simulink model "SMTorqueControl"  (R2026a)
settings: Solver=FixedStepDiscrete  StopTime=1  FixedStep=Ts  EnableMultiTasking=on
PreLoadFcn:
  | if exist(fullfile(pwd, 'Ortak_Veri_ve_Parametreler'), 'dir'), addpath(fullfile(pwd, 'Ortak_Veri_ve_Parametreler')); end
  | if exist(fullfile(pwd, '..', 'Ortak_Veri_ve_Parametreler'), 'dir'), addpath(fullfile(pwd, '..', 'Ortak_Veri_ve_Parametreler')); end
  | if exist(fullfile(pwd, 'Mat_Dosyalari'), 'dir'), addpath(fullfile(pwd, 'Mat_Dosyalari')); end
  | SMTorqueControlData;
InitFcn:
  | if exist(fullfile(pwd, 'Ortak_Veri_ve_Parametreler'), 'dir'), addpath(fullfile(pwd, 'Ortak_Veri_ve_Parametreler')); end
  | if exist(fullfile(pwd, '..', 'Ortak_Veri_ve_Parametreler'), 'dir'), addpath(fullfile(pwd, '..', 'Ortak_Veri_ve_Parametreler')); end
  | if exist(fullfile(pwd, 'Mat_Dosyalari'), 'dir'), addpath(fullfile(pwd, 'Mat_Dosyalari')); end
  | SMTorqueControlData;
undefined symbols (not defined in the file): fsw, Ibase, Ifbase, L_base, Lad, Ld, Lq, p, Tbase, Ts, Tsi, VDC_VECT
libraries: nesl_utility x16, fl_lib x11, ee_lib x6, eeGeneralControl x3, eeTransforms x2, SignalEditorBlockLib x2, eeSmCurrentController x1, eeSmCurrentReferenceGen x1, eePwmGenerator x1, eePwmGeneratorTwoLevel x1, batteryecm_lib x1
Description:
  | SM Torque Control
settings Model: Creator=The MathWorks, Inc.  LastModifiedBy=Dogukan.kilinc
settings DataIOCC: MaxDataPoints=210000  SignalLoggingName=logsout_SMTorqueControl
settings SimscapeCC: SimscapeNominalValues="[{\"value\":\"1\",\"unit\":\"A\"},{\"value\":\"1\",\"unit\":\"bar\"},{\"value\":\"1\",\"unit\":\"cm^2\"},{\"value\":\"1\",\"unit\":\"cm^3/s\"},{\"value\":\"1\",\"unit\":\"kJ/kg\"},{\"value\":\"1\",\"unit\":\"kW\"},{\"value\":\"1\",\"unit\":\"l\"},{\"value\":\"1\",\"unit\":\"N\"},{\"value\":\"1\",\"unit\":\"N*m\"},{\"value\":\"1\",\"unit\":\"V\"}]"  SimscapeLogSimulationStatistics=on  SimscapeLogName=simlog_SMTorqueControl  SimscapeLogDataHistory=210000.0

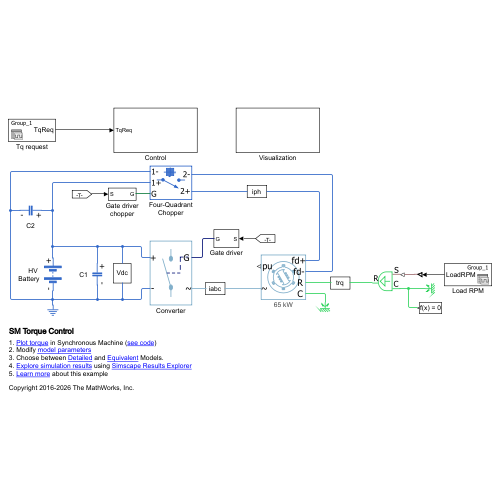
[thumbnail: Simulink's stored preview of the top-level diagram]
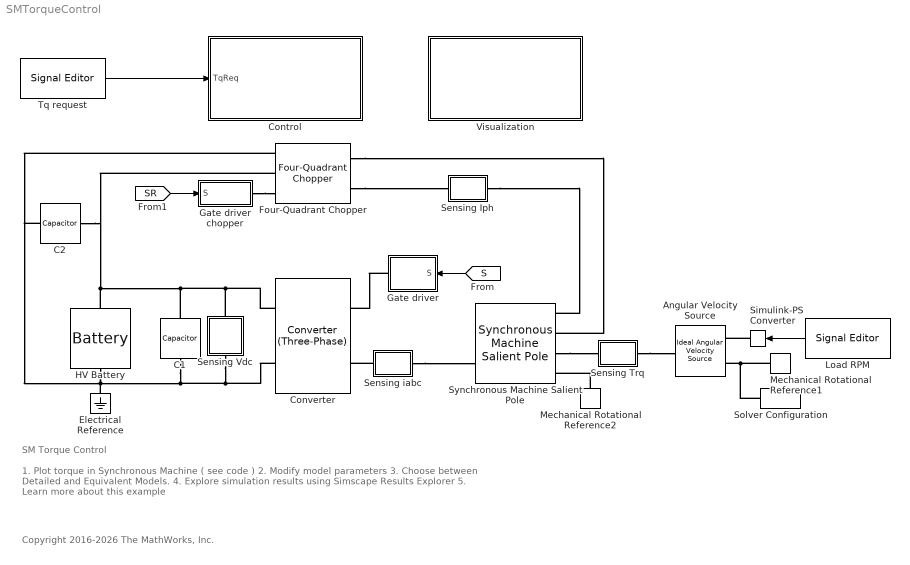
== system SMTorqueControl ==
  note: SM Torque Control
  note: 1. Plot torque in Synchronous Machine ( see code )
      | 2. Modify model parameters
      | 3. Choose between Detailed and Equivalent Models.
      | 4. Explore simulation results using Simscape Results Explorer
      | 5. Learn more about this example
  note: Copyright 2016-2026 The MathWorks, Inc.
  Angular Velocity Source : fl_lib/Mechanical/Mechanical Sources/Ideal Angular Velocity Source
  C1 : fl_lib/Electrical/Electrical Elements/Capacitor  c=Cdc F  r=1e-6 Ohm  g=0 1/Ohm  i_specify=off  i_priority=None  i=0 A  i_nominal_specify=off  i_nominal_value=1  i_nominal_unit=A  v_specify=off  v_priority=None  v=0 V  v_nominal_specify=off  v_nominal_value=1  v_nominal_unit=V  vc_specify=on  vc_priority=None  vc=Vnom V  vc_nominal_specify=off  vc_nominal_value=1  vc_nominal_unit=V
  C2 : fl_lib/Electrical/Electrical Elements/Capacitor  c=Cdc F  r=1e-6 Ohm  g=0 1/Ohm  i_specify=off  i_priority=None  i=0 A  i_nominal_specify=off  i_nominal_value=1  i_nominal_unit=A  v_specify=off  v_priority=None  v=0 V  v_nominal_specify=off  v_nominal_value=1  v_nominal_unit=V  vc_specify=on  vc_priority=None  vc=Vnom V  vc_nominal_specify=off  vc_nominal_value=1  vc_nominal_unit=V
  Control : Subsystem
  Converter : ee_lib/Semiconductors & Converters/Converters/Converter (Three-Phase)  port_option=ee.enum.threePhasePort.composite  fidelity_option=ee.enum.converters.fidelity.detailed  device_type=2  showThermalPort=false  K=0  Vth=0.5 V  Vgt=1 V  Vgt_off=-1 V  Ih=1 A  Vf=0.8 V  Ron=0.001 Ohm  Rds=0.001 Ohm  Goff=1e-5 1/Ohm  Eon_scalar=22.86e-3 J  Eoff_scalar=17.14e-3 J  Eoff_natural_commutation=10e-3 J  Voff=300 V  Iout_scalar=600 A  onCurrentMeasDelay=0 s  useCurrentFromPreviousCycle=false  useVoltageFromPreviousCycle=false  diode_param=2  diode_Vf=0.8 V  diode_Ron=0.001 Ohm  diode_Goff=1e-5 1/Ohm  diode_C=50 nF  diode_iRM=-235 A  diode_iF=300 A  diode_idot=-50 A/us  diode_trr_param=1  diode_trr_factor=3  diode_trr=15 us  diode_Qrr=1.5e+3 s*uA  diode_rec_loss_model=ee.enum.diode.reverseRecoveryModel.fixed  diode_ErecVal=0 J  diode_scaleWithIandV=false  diode_ErecMat=zeros(2, 3) J  diode_TjrecVec=[298.15, 398.15] K  diode_IfrecVec=[.1, 1, 10] A  diode_IrecVal=10 A  diode_VrecVal=10 V  diode_tFilter=1 / 1000 / 100 s  thermal_network_parameterization=ee.enum.thermalNetworkTopology.external  Rth=[.08, .5] K/W  Rth_Cauer=[.08, .1, .5] K/W  Rth_Foster=[.08, .14, .22, .16] K/W  thermal_mass_parameterization=ee.enum.thermalNetwork.timeconstant  thermal_mass=[.01, .5] J/K  thermal_mass_Cauer=[.01, .1, .5] J/K  thermal_mass_Foster=[.001, .005, .05, .5] J/K  thermal_time_constant=[.001, .2] s  thermal_time_constant_Cauer=[.001, .1, .2] s  thermal_time_constant_Foster=[7e-05, .0007, .01, .08] s  thermal_mass_initial_temperatures=[25, 25] degC  thermal_mass_initial_temperatures_Cauer=[25, 25, 25] degC  junction_thermal_mass=0.01 J/K  Tvec_initial_Foster=[25, 25, 25, 25] degC  snubber_type=0  Cs=1e-7 F  Rs=0.1 Ohm  Vce_loss=[0, 150, 300] V
  Electrical Reference : fl_lib/Electrical/Electrical Elements/Electrical Reference
  Four-Quadrant Chopper : ee_lib/Semiconductors & Converters/Converters/Four-Quadrant Chopper  fidelity_option=ee.enum.converters.fidelity.detailed  device_type=3  showThermalPort=false  Vgt=1 V  Vgt_off=-1 V  Ih=1 A  Vf=0.8 V  Ron=0.001 Ohm  Rds=0.001 Ohm  Goff=1e-5 1/Ohm  Vth=0.5 V  K=0  Eon_scalar=22.86e-3 J  Eoff_scalar=17.14e-3 J  Eoff_natural_commutation=10e-3 J  Voff=300 V  Iout_scalar=600 A  onCurrentMeasDelay=0 s  useCurrentFromPreviousCycle=false  useVoltageFromPreviousCycle=false  diode_param=2  diode_Vf=0.8 V  diode_Ron=0.001 Ohm  diode_Goff=1e-5 1/Ohm  diode_C=50 nF  diode_iRM=-235 A  diode_iF=300 A  diode_idot=-50 A/us  diode_trr_param=1  diode_trr_factor=3  diode_trr=15 us  diode_Qrr=1500 s*uA  diode_rec_loss_model=ee.enum.diode.reverseRecoveryModel.fixed  diode_ErecVal=0 J  diode_scaleWithIandV=false  diode_ErecMat=zeros(2, 3) J  diode_TjrecVec=[298.15, 398.15] K  diode_IfrecVec=[.1, 1, 10] A  diode_IrecVal=10 A  diode_VrecVal=10 V  diode_tFilter=1 / 1000 / 100 s  thermal_network_parameterization=ee.enum.thermalNetworkTopology.external  Rth=[.08, .5] K/W  Rth_Cauer=[.08, .1, .5] K/W  Rth_Foster=[.08, .14, .22, .16] K/W  thermal_mass_parameterization=ee.enum.thermalNetwork.timeconstant  thermal_mass=[.01, .5] J/K  thermal_mass_Cauer=[.01, .1, .5] J/K  thermal_mass_Foster=[.001, .005, .05, .5] J/K  thermal_time_constant=[.001, .2] s  thermal_time_constant_Cauer=[.001, .1, .2] s  thermal_time_constant_Foster=[7e-05, .0007, .01, .08] s  thermal_mass_initial_temperatures=[25, 25] degC  thermal_mass_initial_temperatures_Cauer=[25, 25, 25] degC  junction_thermal_mass=0.01 J/K  Tvec_initial_Foster=[25, 25, 25, 25] degC  snubber_type=0  Cs=1e-7 F  Rs=0.1 Ohm
  Gate driver : Subsystem
  Gate driver chopper : Subsystem
  HV Battery : batteryecm_lib/Battery  Vnom=Vnom V  prm_dir=1  R1_dis=2 Ohm  R1_ch=2 Ohm  R1=0.001 Ohm  prm_AH=1  AH=300 hr*A  V1=330 V  AH1=100 hr*A  prm_R2=1  R2=2000 Ohm  Tmeas=298.15 K  charge_measurement_port=simscape.enum.battery.enable.no  prm_dyn=1  Rp1=0.005 Ohm  tau1=30 s  Rp2=0.005 Ohm  tau2=30 s  Rp3=0.005 Ohm  tau3=30 s  Rp4=0.005 Ohm  tau4=30 s  Rp5=0.005 Ohm  tau5=30 s  prm_fade=1  N_fade=100  AH_fade=45 hr*A  R1_fade=2.02 Ohm  R1_ch_fade=2.02 Ohm  V1_fade=10.35 V  prm_age=1  prm_age_OCV=1  OCV_age=0.9  SOC_age=60  Tmeas_age=298.15 K  delta_time_age_vec=[0] d  temperature_age_vec=[273] K  OCV_scaling_age=2.2134e6  OCV_offset_age=1.632e6  temp_exp_age=0.515833569 V  t_exp_age=0.75  Vnom_T2=12 V  R1_T2=2.2 Ohm  R1_T2_dis=2.2 Ohm  R1_T2_ch=2.2 Ohm  V1_T2=11.4 V  R2_T2=2200 Ohm  Rp1_T2=0.005 Ohm  tau1_T2=30 s  Rp2_T2=0.005 Ohm  tau2_T2=30 s  Rp3_T2=0.005 Ohm  tau3_T2=30 s  Rp4_T2=0.005 Ohm  tau4_T2=30 s  Rp5_T2=0.005 Ohm  tau5_T2=30 s  Tmeas2=273.15 K  thermal_port=simscape.enum.thermaleffects.omit  thermal_mass=30000 J/K  i_specify=off  i_priority=None  i=0 A  i_nominal_specify=off  i_nominal_value=1  i_nominal_unit=A  v_specify=off  v_priority=None  v=0 V  v_nominal_specify=off  v_nominal_value=1  v_nominal_unit=V  charge_specify=on  charge_priority=High  charge=AH0 hr*A  charge_nominal_specify=off  charge_nominal_value=1  charge_nominal_unit=A*hr  num_cycles_specify=off  num_cycles_priority=High  num_cycles=0  num_cycles_nominal_specify=off  num_cycles_nominal_value=1  num_cycles_nominal_unit=1  temperature_specify=off  temperature_priority=High  temperature=298.15 K  temperature_nominal_specify=off  temperature_nominal_value=1  temperature_nominal_unit=K
  Load RPM : SignalEditorBlockLib/Signal Editor  FileName=SMTorqueControlLoadRPM.mat  ActiveScenario=Group_1  ActiveSignal=LoadRPM  IsBus=off  OutputBusObjectStr=Bus: BusObject  SampleTime=0  OutputAfterFinalValue=Extrapolation  Unit=inherit  PreserveSignalName=on  ApplySigPropsToAllScenarios=on  ApplySigPropsToAllSignals=off  SignalPropertySource=Dialog parameters
  Mechanical Rotational Reference1 : fl_lib/Mechanical/Rotational Elements/Mechanical Rotational Reference
  Mechanical Rotational Reference2 : fl_lib/Mechanical/Rotational Elements/Mechanical Rotational Reference
  Sensing Iph : Subsystem
      mask Display: disp('iph')
  Sensing Trq : Subsystem
      mask Display: disp('trq')
  Sensing Vdc : Subsystem
      mask Display: disp('Vdc')
  Sensing iabc : Subsystem
      mask Display: disp('iabc')
  Simulink-PS Converter : nesl_utility/Simulink-PS Converter  PhysicalDomain=network_engine_domain  SubClassName=ps_input  LeftPortType=input  RightPortType=output  PseudoPeriodic=off  Frequencies=[]  NoiseDistribution=none  NoiseParameters=[]  Unit=rpm  AffineConversion=off  FilteringAndDerivatives=zero  SimscapeFilterOrder=1  InputFilterTimeConstant=0.001  UdotUserProvided=1
  Solver Configuration : nesl_utility/Solver Configuration  PhysicalDomain=network_engine_domain  SubClassName=solver  LeftPortType=input  RightPortType=generic  Tones=[]  Harmonics=[]  SimulateNoise=off  Profile=off  UseLocalSampling=off  EnableSwitchedLinearOptims=on  FrequencyDomain=off  UseCCode=off  RelTol=0.001  AbsTol=1e-06  MinStep=1e-09  ToWorkspace=off  RevertToSquareIcSolve=off  NumHomotopyIterations=100  PhasorMode=off  PhasorModeNumHarmonics=1  ConsistencySolver=NEWTON_FTOL  CanonicalOrdering=UNORDERED  OptimizeIntermediates=UNOPTIMIZED  IndexReductionMethod=DerivativeReplacement  DoDC=off  ResidualTolerance=1e-9  ConsistencyTolSource=GLOBAL  ConsistencyAbsTol=0.001  ConsistencyRelTol=0.001  ConsistencyTolFactor=0.001  UseLocalSolver=on  LocalSolverChoice=NE_BACKWARD_EULER_ADVANCER  ResolveIndetEquations=on  FunctionEvalNumThread=1  LocalSolverSampleTime=Ts  DoFixedCost=on  MaxNonlinIter=4  MaxModeIter=2  ComputeImpulses=off  ImpulseIterations=2  LinearAlgebra=auto  LinearAlgebraNumThread=0  EquationFormulation=NE_TIME_EF  DelaysMemoryBudget=1024  AutomaticFiltering=on  FilteringTimeConstant=0.001  PartitionStorageMethod=AS_NEEDED  PartitionMemoryBudget=1024  PartitionMethod=FAST  MultibodyUseLocalSolver=off  MultibodyLocalSolverChoice=ODE1  MultibodyLocalSolverSampleTime=0.001
  Synchronous Machine Salient Pole : ee_lib/Electromechanical/Synchronous/Synchronous Machine Salient Pole  port_option=ee.enum.threePhasePort.composite  SRated=Pmax W  VRated=Vr V  FRated=fr Hz  nPolePairs=p  param_option=ee.enum.sm.parameterization.fundamental  fieldCircuitParameterization_option=2  baseEfd=272 V  baseIfd=Ifbase A  zero_sequence=ee.enum.park.zerosequence.exclude  axes_param=ee.enum.rotorangle.daxis  Ladu=Lad  Laqu=Laq  L0=L0  Ll=Ll  Ra=Rs  Lfd=Lfd  Rfd=Rfd  L1d=0.1  R1d=0.254  L1q=0.1567  R1q=0.328  Xl=0.15  Xd=1.05  Xq=0.7  X0=0.15  Xdd=0.35  Xddd=0.25  Xqdd=0.325  d_option=ee.enum.circuit.open  Td0d=5.25 s  Tdd=1.75 s  Td0dd=0.03 s  Tddd=0.0214 s  q_option=ee.enum.circuit.open  Tq0dd=0.05 s  Tqdd=0.0232 s  saturation_option=0  saturation_ifd=[0.0, 0.48, 0.76, 1.38, 1.79]  saturation_Vag=[0.0, 0.43, 0.59, 0.71, 0.76]  initialization_option=1  source_type=ee.enum.sm.load_flow_source_type.Swing  Vmag0=Vr V  Vang0=0 deg  Pt0=0 V*A  Qt0=0 V*A  minimum_pu=0.95  phase_search_range=[-30, 30] deg  gmin=1e-6 S  connection_option=ee.enum.Connection.wye  num_q_dampers=1  rotor_offset=-pi / 2 rad  pu_psid_specify=on  pu_psid_priority=High  pu_psid=0  pu_psid_nominal_specify=off  pu_psid_nominal_value=1  pu_psid_nominal_unit=1  pu_psiq_specify=on  pu_psiq_priority=High  pu_psiq=0  pu_psiq_nominal_specify=off  pu_psiq_nominal_value=1  pu_psiq_nominal_unit=1  pu_psifd_specify=on  pu_psifd_priority=High  pu_psifd=0  pu_psifd_nominal_specify=off  pu_psifd_nominal_value=1  pu_psifd_nominal_unit=1  pu_psi1d_specify=on  pu_psi1d_priority=High  pu_psi1d=0  pu_psi1d_nominal_specify=off  pu_psi1d_nominal_value=1  pu_psi1d_nominal_unit=1  pu_psi1q_specify=on  pu_psi1q_priority=High  pu_psi1q=0  pu_psi1q_nominal_specify=off  pu_psi1q_nominal_value=1  pu_psi1q_nominal_unit=1  angular_position_diff_specify=on  angular_position_diff_priority=High  angular_position_diff=-pi/2/p rad  angular_position_diff_nominal_specify=off  angular_position_diff_nominal_value=1  angular_position_diff_nominal_unit=deg  Tmeas=298.15 K  alpha=3.93e-3 1/K  stator_thermal_mass=100 J/K  rotor_thermal_mass=200 J/K  temperatureA_specify=off  temperatureA_priority=High  temperatureA=25 degC  temperatureA_nominal_specify=off  temperatureA_nominal_value=1  temperatureA_nominal_unit=degC  temperatureB_specify=off  temperatureB_priority=High  temperatureB=25 degC  temperatureB_nominal_specify=off  temperatureB_nominal_value=1  temperatureB_nominal_unit=degC  temperatureC_specify=off  temperatureC_priority=High  temperatureC=25 degC  temperatureC_nominal_specify=off  temperatureC_nominal_value=1  temperatureC_nominal_unit=degC  temperatureR_specify=off  temperatureR_priority=High  temperatureR=25 degC  temperatureR_nominal_specify=off  temperatureR_nominal_value=1  temperatureR_nominal_unit=degC
      settings: AttributesFormatString=65 kW
  Tq request : SignalEditorBlockLib/Signal Editor  FileName=SMTorqueControlTorqueRequest.mat  ActiveScenario=Group_1  ActiveSignal=TqReq  IsBus=off  OutputBusObjectStr=Bus: BusObject  SampleTime=0  OutputAfterFinalValue=Extrapolation  Unit=inherit  PreserveSignalName=on  ApplySigPropsToAllScenarios=on  ApplySigPropsToAllSignals=off  SignalPropertySource=Dialog parameters
  Visualization : Subsystem
  wires:
  [S] -> Gate driver/1(S)
  Load RPM/1 -> Simulink-PS Converter/1
  [SR] -> Gate driver chopper/1(S)
  Tq request/1 -> Control/1(TqReq)
  connections:
  Sensing Trq/RConn1 -- Angular Velocity Source/LConn1
  Converter/RConn2 -- Sensing Vdc/RConn1 -- Four-Quadrant Chopper/LConn3 -- C2/RConn1 -- HV Battery/RConn1 -- Electrical Reference/LConn1 -- C1/RConn1
  Converter/RConn1 -- Sensing Vdc/LConn1 -- Four-Quadrant Chopper/LConn2 -- C2/LConn1 -- HV Battery/LConn1 -- C1/LConn1
  Gate driver/RConn1 -- Converter/LConn1
  Simulink-PS Converter/RConn1 -- Angular Velocity Source/RConn1
  Synchronous Machine Salient Pole/LConn3 -- Sensing Trq/LConn1
  Mechanical Rotational Reference1/LConn1 -- Solver Configuration/RConn1 -- Angular Velocity Source/RConn2
  Four-Quadrant Chopper/RConn1 -- Sensing Iph/LConn1
  Four-Quadrant Chopper/RConn2 -- Synchronous Machine Salient Pole/LConn2
  Sensing Iph/RConn1 -- Synchronous Machine Salient Pole/LConn1
  Sensing iabc/LConn1 -- Converter/LConn2
  Sensing iabc/RConn1 -- Synchronous Machine Salient Pole/RConn2
  Gate driver chopper/RConn1 -- Four-Quadrant Chopper/LConn1
  Mechanical Rotational Reference2/LConn1 -- Synchronous Machine Salient Pole/LConn4

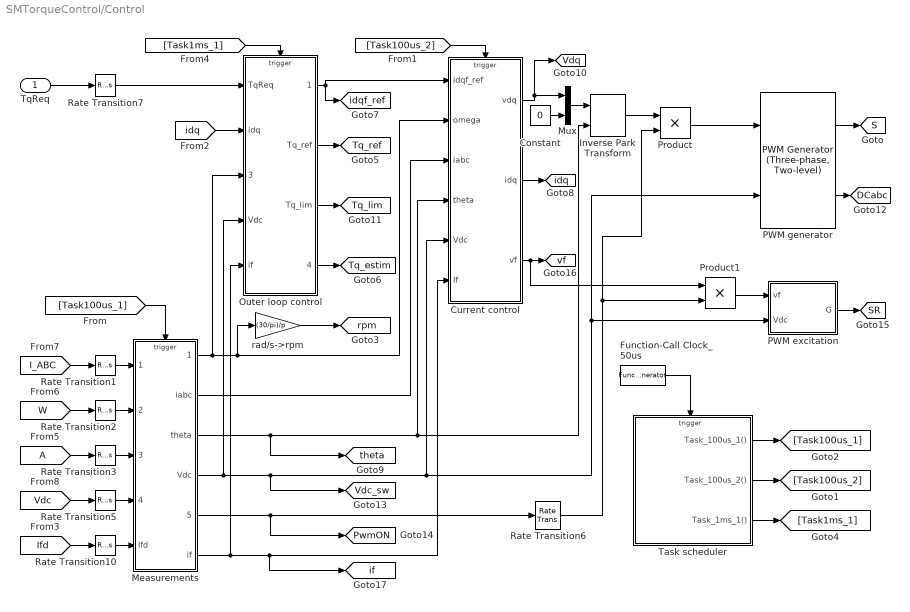
== system SMTorqueControl/Control ==
  TqReq : Inport
  Constant : Constant  Value=0  SampleTime=-1
  Current control : Subsystem
  From5 : From  TagVisibility=global
  Function-Call Clock_50us : FunctionCallGenerator  SampleTime=5e-5
  Inverse Park Transform : eeTransforms/Inverse Park Transform  AxisAlignment=Q-axis  PowerInvariant=off
  Measurements : Subsystem
  Mux : Mux  Inputs=2
  Outer loop control : Subsystem
  PWM excitation : Subsystem
  PWM generator : eePwmGeneratorTwoLevel/PWM Generator (Three-phase, Two-level)  PWMMode=Continuous PWM (CPWM)  CPWMMode=SVM: space vector modulation  DPWMMode=60 DPWM: 60 degree discontinuous PWM  fsw=fsw  Ts=Ts
  Product : Product
  Product1 : Product
  Rate Transition{1..3,5..7,10} (7 alike) : RateTransition
  Task scheduler : Stateflow chart  TreatAsAtomicUnit=on
  rad/s->rpm : Gain  Gain=(30/pi)/p
  tag scope: DCabc=global, PwmON=global, S=global, SR=global, Tq_estim=global, Tq_lim=global, Tq_ref=global, Vdc_sw=global, Vdq=global, idq=global, idqf_ref=global, if=global, rpm=global, theta=global, vf=global
  wires:
  [Ifd] -> Rate Transition10/1
  [W] -> Rate Transition2/1
  [idq] -> Outer loop control/2(idq)
  [Task100us_1] -> Measurements/Trigger
  Measurements/5(PwmON) -> Rate Transition6/1, [PwmON]
  Rate Transition1/1 -> Measurements/1(iabc_m)
  PWM generator/2 -> [DCabc]
  [I_ABC] -> Rate Transition1/1
  Rate Transition6/1 -> Product1/2, Product/2
  [Task100us_2] -> Current control/Trigger
  Measurements/2(iabc) -> Current control/3(iabc)
  Outer loop control/4(Tq_estim) -> [Tq_estim]
  Current control/3(vf) -> Product1/1, [vf]
  Measurements/1(omega) -> rad/s->rpm/1, Current control/2(omega), Outer loop control/3(omega)
  rad/s->rpm/1 -> [rpm]
  Current control/2(idq) -> [idq]
  Rate Transition10/1 -> Measurements/5(Ifd)
  Task scheduler/2(Task_100us_2()) -> [Task100us_2]
  From5/1 -> Rate Transition3/1
  Measurements/3(theta) -> [theta], Inverse Park Transform/2, Current control/4(theta)
  Outer loop control/2(Tq_ref) -> [Tq_ref]
  Task scheduler/1(Task_100us_1()) -> [Task100us_1]
  [Task1ms_1] -> Outer loop control/Trigger
  Rate Transition2/1 -> Measurements/2(omega_m)
  Task scheduler/3(Task_1ms_1()) -> [Task1ms_1]
  TqReq/1 -> Rate Transition7/1
  Measurements/4(Vdc) -> [Vdc_sw], PWM generator/2, PWM excitation/2(Vdc), Current control/5(Vdc), Outer loop control/4(Vdc)
  [Vdc] -> Rate Transition5/1
  Rate Transition5/1 -> Measurements/4(Vdc_m)
  PWM generator/1 -> [S]
  Rate Transition3/1 -> Measurements/3(theta_m)
  Outer loop control/3(Tq_lim) -> [Tq_lim]
  Measurements/6(if) -> [if], Current control/6(If), Outer loop control/5(if)
  PWM excitation/1(G) -> [SR]
  Function-Call Clock_50us/1 -> Task scheduler/Trigger
  Rate Transition7/1 -> Outer loop control/1(TqReq)
  Outer loop control/1(idqf_ref) -> Current control/1(idqf_ref), [idqf_ref]
  Constant/1 -> Mux/2
  Mux/1 -> Inverse Park Transform/1
  Current control/1(vdq) -> [Vdq], Mux/1
  Product/1 -> PWM generator/1
  Inverse Park Transform/1 -> Product/1
  Product1/1 -> PWM excitation/1(vf)

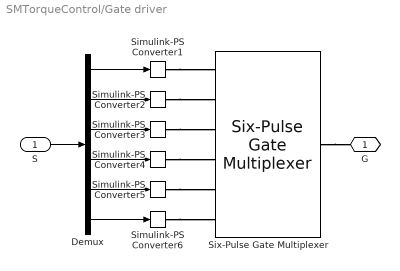
== system SMTorqueControl/Gate driver ==
  S : Inport
  Demux : Demux  Outputs=6
  Simulink-PS Converter{1..6} (6 alike) : nesl_utility/Simulink-PS Converter  PhysicalDomain=network_engine_domain  SubClassName=ps_input  LeftPortType=input  RightPortType=output  PseudoPeriodic=off  Frequencies=[]  NoiseDistribution=none  NoiseParameters=[]  Unit=1  AffineConversion=off  FilteringAndDerivatives=zero  SimscapeFilterOrder=1  InputFilterTimeConstant=0.001  UdotUserProvided=1
  Six-Pulse Gate Multiplexer : ee_lib/Semiconductors & Converters/Converters/Six-Pulse Gate Multiplexer  port_option=ee.enum.controlport.ps
  G : PMIOPort  Side=Right
  wires:
  Demux/1 -> Simulink-PS Converter1/1
  S/1 -> Demux/1
  Demux/4 -> Simulink-PS Converter4/1
  Demux/2 -> Simulink-PS Converter2/1
  Demux/3 -> Simulink-PS Converter3/1
  Demux/5 -> Simulink-PS Converter5/1
  Demux/6 -> Simulink-PS Converter6/1
  connections:
  Six-Pulse Gate Multiplexer/RConn1 -- G/RConn1
  Simulink-PS Converter1/RConn1 -- Six-Pulse Gate Multiplexer/LConn1
  Simulink-PS Converter3/RConn1 -- Six-Pulse Gate Multiplexer/LConn3
  Simulink-PS Converter5/RConn1 -- Six-Pulse Gate Multiplexer/LConn5
  Simulink-PS Converter6/RConn1 -- Six-Pulse Gate Multiplexer/LConn6
  Simulink-PS Converter4/RConn1 -- Six-Pulse Gate Multiplexer/LConn4
  Simulink-PS Converter2/RConn1 -- Six-Pulse Gate Multiplexer/LConn2

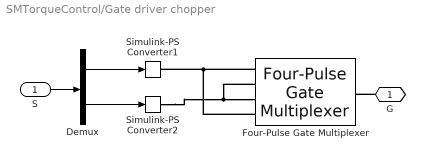
== system SMTorqueControl/Gate driver chopper ==
  S : Inport
  Demux : Demux  Outputs=2
  Four-Pulse Gate Multiplexer : ee_lib/Semiconductors & Converters/Converters/Four-Pulse Gate Multiplexer  port_option=ee.enum.controlport.ps
  Simulink-PS Converter1 : nesl_utility/Simulink-PS Converter  PhysicalDomain=network_engine_domain  SubClassName=ps_input  LeftPortType=input  RightPortType=output  PseudoPeriodic=off  Frequencies=[]  NoiseDistribution=none  NoiseParameters=[]  Unit=1  AffineConversion=off  FilteringAndDerivatives=zero  SimscapeFilterOrder=1  InputFilterTimeConstant=0.001  UdotUserProvided=1
  Simulink-PS Converter2 : nesl_utility/Simulink-PS Converter  PhysicalDomain=network_engine_domain  SubClassName=ps_input  LeftPortType=input  RightPortType=output  PseudoPeriodic=off  Frequencies=[]  NoiseDistribution=none  NoiseParameters=[]  Unit=1  AffineConversion=off  FilteringAndDerivatives=zero  SimscapeFilterOrder=1  InputFilterTimeConstant=0.001  UdotUserProvided=1
  G : PMIOPort  Side=Right
  wires:
  Demux/2 -> Simulink-PS Converter2/1
  S/1 -> Demux/1
  Demux/1 -> Simulink-PS Converter1/1
  connections:
  Simulink-PS Converter2/RConn1 -- Four-Pulse Gate Multiplexer/LConn2 -- Four-Pulse Gate Multiplexer/LConn3
  Four-Pulse Gate Multiplexer/LConn1 -- Four-Pulse Gate Multiplexer/LConn4 -- Simulink-PS Converter1/RConn1
  G/RConn1 -- Four-Pulse Gate Multiplexer/RConn1

== system SMTorqueControl/Sensing Iph ==
  Current Sensor : fl_lib/Electrical/Electrical Sensors/Current Sensor
  PS-Simulink Converter : nesl_utility/PS-Simulink Converter  PhysicalDomain=network_engine_domain  SubClassName=ps_output  LeftPortType=input  RightPortType=output  PseudoPeriodic=off  Frequencies=[]  VectorFormat=1-D array  Unit=1  AffineConversion=off
  + : PMIOPort  Side=Left
  - : PMIOPort  Port=2  Side=Right
  tag scope: Ifd=global
  wires:
  PS-Simulink Converter/1 -> [Ifd]
  connections:
  Current Sensor/LConn1 -- +/RConn1
  Current Sensor/RConn2 -- -/RConn1
  PS-Simulink Converter/LConn1 -- Current Sensor/RConn1

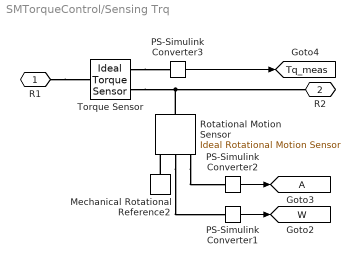
== system SMTorqueControl/Sensing Trq ==
  Goto3 : Goto  TagVisibility=global
  Mechanical Rotational Reference2 : fl_lib/Mechanical/Rotational Elements/Mechanical Rotational Reference
  PS-Simulink Converter1 : nesl_utility/PS-Simulink Converter  PhysicalDomain=network_engine_domain  SubClassName=ps_output  LeftPortType=input  RightPortType=output  PseudoPeriodic=off  Frequencies=[]  VectorFormat=1-D array  Unit=rad/s  AffineConversion=off
  PS-Simulink Converter2 : nesl_utility/PS-Simulink Converter  PhysicalDomain=network_engine_domain  SubClassName=ps_output  LeftPortType=input  RightPortType=output  PseudoPeriodic=off  Frequencies=[]  VectorFormat=1-D array  Unit=rad  AffineConversion=off
  PS-Simulink Converter3 : nesl_utility/PS-Simulink Converter  PhysicalDomain=network_engine_domain  SubClassName=ps_output  LeftPortType=input  RightPortType=output  PseudoPeriodic=off  Frequencies=[]  VectorFormat=1-D array  Unit=N*m  AffineConversion=off
  Rotational Motion Sensor : fl_lib/Mechanical/Mechanical Sensors/Ideal Rotational Motion Sensor  reference=foundation.enum.MeasurementReference.difference  acceleration_port=false  velocity_port=true  position_port=true  wrap_angle=simscape.enum.onoff.off  offset=0 deg
  Torque Sensor : fl_lib/Mechanical/Mechanical Sensors/Ideal Torque Sensor
  R1 : PMIOPort  Side=Left
  R2 : PMIOPort  Port=2  Side=Right
  tag scope: Tq_meas=global, W=global
  wires:
  PS-Simulink Converter1/1 -> [W]
  PS-Simulink Converter2/1 -> Goto3/1
  PS-Simulink Converter3/1 -> [Tq_meas]
  connections:
  Rotational Motion Sensor/LConn1 -- Torque Sensor/RConn1 -- R2/RConn1
  Torque Sensor/RConn2 -- PS-Simulink Converter3/LConn1
  Rotational Motion Sensor/RConn2 -- PS-Simulink Converter1/LConn1
  Rotational Motion Sensor/RConn3 -- PS-Simulink Converter2/LConn1
  Mechanical Rotational Reference2/LConn1 -- Rotational Motion Sensor/RConn1
  R1/RConn1 -- Torque Sensor/LConn1

== system SMTorqueControl/Sensing Vdc ==
  PS-Simulink Converter4 : nesl_utility/PS-Simulink Converter  PhysicalDomain=network_engine_domain  SubClassName=ps_output  LeftPortType=input  RightPortType=output  PseudoPeriodic=off  Frequencies=[]  VectorFormat=1-D array  Unit=V  AffineConversion=off
  Voltage Sensor : fl_lib/Electrical/Electrical Sensors/Voltage Sensor
  + : PMIOPort  Side=Left
  - : PMIOPort  Port=2  Side=Right
  tag scope: Vdc=global
  wires:
  PS-Simulink Converter4/1 -> [Vdc]
  connections:
  Voltage Sensor/LConn1 -- +/RConn1
  Voltage Sensor/RConn2 -- -/RConn1
  PS-Simulink Converter4/LConn1 -- Voltage Sensor/RConn1

== system SMTorqueControl/Sensing iabc ==
  Current Sensor : ee_lib/Sensors & Transducers/Current Sensor (Three-Phase)  port_option=ee.enum.threePhasePort.composite
  PS-Simulink Converter : nesl_utility/PS-Simulink Converter  PhysicalDomain=network_engine_domain  SubClassName=ps_output  LeftPortType=input  RightPortType=output  PseudoPeriodic=off  Frequencies=[]  VectorFormat=1-D array  Unit=A  AffineConversion=off
  1 : PMIOPort  Side=Left
  2 : PMIOPort  Port=2  Side=Right
  tag scope: I_ABC=global
  wires:
  PS-Simulink Converter/1 -> [I_ABC]
  connections:
  1/RConn1 -- Current Sensor/LConn1
  2/RConn1 -- Current Sensor/RConn2
  Current Sensor/RConn1 -- PS-Simulink Converter/LConn1

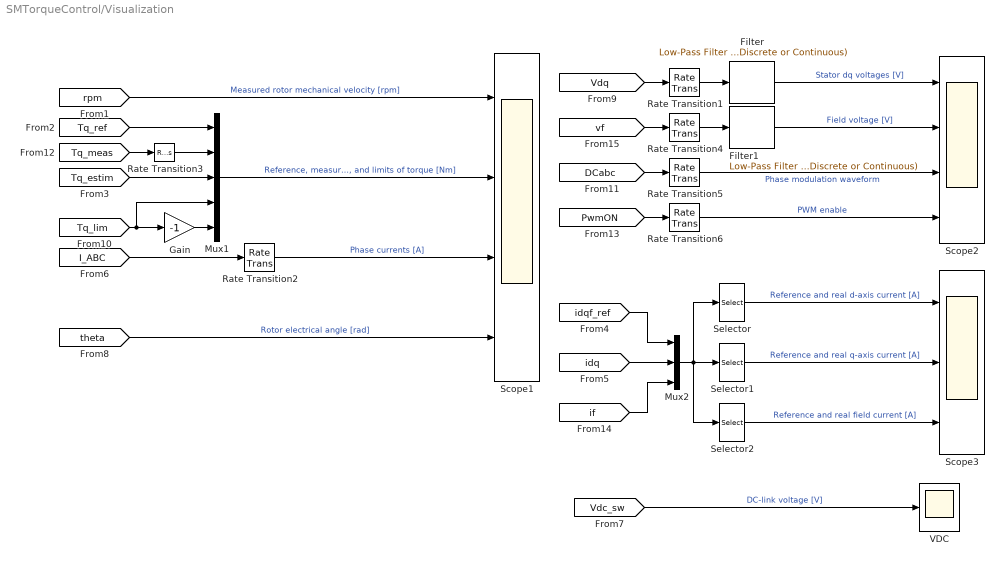
== system SMTorqueControl/Visualization ==
  Filter : eeGeneralControl/Low-Pass Filter (Discrete or Continuous)  K=1  T=0.05  B=inf  A=-inf  init_option=Inherited from block input  x0=0  Ts=Tsi
  Filter1 : eeGeneralControl/Low-Pass Filter (Discrete or Continuous)  K=1  T=0.05  B=inf  A=-inf  init_option=Inherited from block input  x0=0  Ts=Tsi
  Gain : Gain  Gain=-1
  Mux1 : Mux  Inputs=5
  Mux2 : Mux  Inputs=3
  Rate Transition{1,4..6} (4 alike) : RateTransition  OutPortSampleTime=Tsi
  Rate Transition2 : RateTransition
  Rate Transition3 : RateTransition
  Scope1 : Scope  NumInputPorts=4
      settings: ActiveDisplayYMinimum=-250  ActiveDisplayYMaximum=2250  DataLoggingSaveFormat=Array
  Scope2 : Scope  NumInputPorts=4
      settings: ActiveDisplayYMinimum=-110.23475  ActiveDisplayYMaximum=89.83125  DataLoggingVariableName=ScopeData3  DataLoggingSaveFormat=Array
  "Scope3 " : Scope  NumInputPorts=3
      settings: ActiveDisplayYMinimum=-147.62964  ActiveDisplayYMaximum=49.34388  DataLoggingVariableName=ScopeData2  DataLoggingSaveFormat=Array
  Selector : Selector  InputPortWidth=6  IndexOptions=Index vector (dialog)  Indices=[1 4]  OutputSizes=1
  Selector1 : Selector  InputPortWidth=6  IndexOptions=Index vector (dialog)  Indices=[2 5]  OutputSizes=1
  Selector2 : Selector  InputPortWidth=6  IndexOptions=Index vector (dialog)  Indices=[3 6]  OutputSizes=1
  VDC : Scope
      settings: ActiveDisplayYMinimum=-43.65366  ActiveDisplayYMaximum=392.90021  DataLoggingSaveFormat=Array
  wires:
  [if] -> Mux2/3
  Filter/1 -> Scope2/1  "Stator dq voltages [V]"
  [DCabc] -> Rate Transition5/1
  Rate Transition3/1 -> Mux1/2
  [Tq_ref] -> Mux1/1
  [Vdc_sw] -> VDC/1  "DC-link voltage [V]"
  [PwmON] -> Rate Transition6/1
  [rpm] -> Scope1/1  "Measured rotor mechanical velocity [rpm]"
  [Tq_meas] -> Rate Transition3/1
  Rate Transition2/1 -> Scope1/3  "Phase currents [A]"
  Mux2/1 -> Selector/1, Selector2/1, Selector1/1
  [Tq_estim] -> Mux1/3
  [idqf_ref] -> Mux2/1
  [idq] -> Mux2/2
  [Tq_lim] -> Gain/1, Mux1/4
  Filter1/1 -> Scope2/2  "Field voltage [V]"
  [theta] -> Scope1/4  "Rotor electrical angle [rad]"
  Gain/1 -> Mux1/5
  [I_ABC] -> Rate Transition2/1
  Mux1/1 -> Scope1/2  "Reference, measured, estim, and limits of torque [Nm]"
  Selector1/1 -> "Scope3 "/2  "Reference and real q-axis current [A]"
  Selector/1 -> "Scope3 "/1  "Reference and real d-axis current [A]"
  Selector2/1 -> "Scope3 "/3  "Reference and real field current [A]"
  Rate Transition4/1 -> Filter1/1
  Rate Transition1/1 -> Filter/1
  [Vdq] -> Rate Transition1/1
  [vf] -> Rate Transition4/1
  Rate Transition5/1 -> Scope2/3  "Phase modulation waveform"
  Rate Transition6/1 -> Scope2/4  "PWM enable"

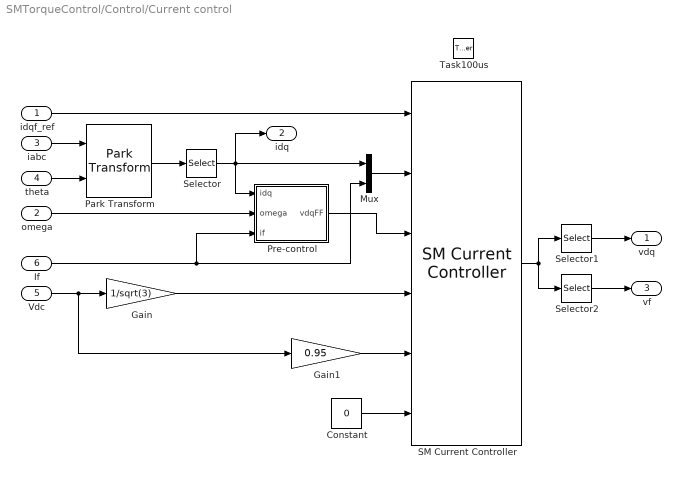
== system SMTorqueControl/Control/Current control ==
  idqf_ref : Inport
  omega : Inport  Port=2
  iabc : Inport  Port=3
  theta : Inport  Port=4
  Vdc : Inport  Port=5
  If : Inport  Port=6
  Task100us : TriggerPort  TriggerType=function-call  VariantControl=Variant  PortDimensions=1
  Constant : Constant  Value=0  SampleTime=-1
  Gain : Gain  Gain=1/sqrt(3)
  Gain1 : Gain  Gain=0.95
  Mux : Mux  Inputs=2
  Park Transform : eeTransforms/Park Transform  AxisAlignment=Q-axis  PowerInvariant=off
  Pre-control : Subsystem
  SM Current Controller : eeSmCurrentController/SM Current Controller  Ts=-1  Tsd=Tsi  AxisPrio=Q-axis  ActZC=on  ActFF=on  Kp_id=Kp_id  Ki_id=Ki_id  Kaw_id=Kaw_id  Kp_iq=Kp_iq  Ki_iq=Ki_iq  Kaw_iq=Kaw_iq  Kp_if=Kp_if  Ki_if=Ki_if  Kaw_if=Kaw_if
  Selector : Selector  InputPortWidth=3  IndexOptions=Index vector (dialog)  Indices=[1 2]  OutputSizes=1
  Selector1 : Selector  InputPortWidth=3  IndexOptions=Index vector (dialog)  Indices=[1 2]  OutputSizes=1
  Selector2 : Selector  InputPortWidth=3  IndexOptions=Index vector (dialog)  Indices=3  OutputSizes=1
  vdq : Outport  VectorParamsAs1DForOutWhenUnconnected=off
  idq : Outport  Port=2  VectorParamsAs1DForOutWhenUnconnected=off
  vf : Outport  Port=3  VectorParamsAs1DForOutWhenUnconnected=off
  wires:
  iabc/1 -> Park Transform/1
  Park Transform/1 -> Selector/1
  theta/1 -> Park Transform/2
  idqf_ref/1 -> SM Current Controller/1
  Selector/1 -> Mux/1, idq/1, Pre-control/1(idq)
  Pre-control/1(vdqFF) -> SM Current Controller/3
  Vdc/1 -> Gain1/1, Gain/1
  omega/1 -> Pre-control/2(omega)
  If/1 -> Pre-control/3(if), Mux/2
  Gain/1 -> SM Current Controller/4
  Gain1/1 -> SM Current Controller/5
  Constant/1 -> SM Current Controller/6
  SM Current Controller/1 -> Selector2/1, Selector1/1
  Selector1/1 -> vdq/1
  Selector2/1 -> vf/1
  Mux/1 -> SM Current Controller/2

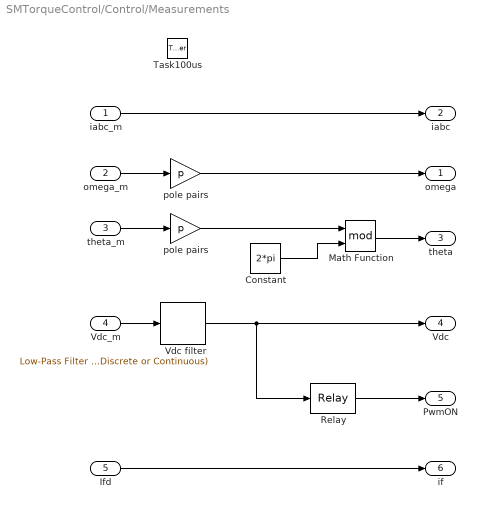
== system SMTorqueControl/Control/Measurements ==
  iabc_m : Inport
  omega_m : Inport  Port=2
  theta_m : Inport  Port=3
  Vdc_m : Inport  Port=4
  Ifd : Inport  Port=5
  Task100us : TriggerPort  TriggerType=function-call  VariantControl=Variant  PortDimensions=1
  Constant : Constant  Value=2*pi  SampleTime=-1
  Math Function : Math  Operator=mod  SignedPower=on
  Relay : Relay  OnSwitchValue=VDC_VECT(1)  OffSwitchValue=0.5*VDC_VECT(1)
  Vdc filter : eeGeneralControl/Low-Pass Filter (Discrete or Continuous)  K=1  T=0.005  B=inf  A=-inf  init_option=Inherited from block input  x0=0  Ts=-1
  pole pairs : Gain  Gain=p
  "pole pairs " : Gain  Gain=p
  omega : Outport  VectorParamsAs1DForOutWhenUnconnected=off
  iabc : Outport  Port=2  VectorParamsAs1DForOutWhenUnconnected=off
  theta : Outport  Port=3  VectorParamsAs1DForOutWhenUnconnected=off
  Vdc : Outport  Port=4  VectorParamsAs1DForOutWhenUnconnected=off
  PwmON : Outport  Port=5  VectorParamsAs1DForOutWhenUnconnected=off
  if : Outport  Port=6  VectorParamsAs1DForOutWhenUnconnected=off
  wires:
  pole pairs/1 -> omega/1
  Vdc_m/1 -> Vdc filter/1
  theta_m/1 -> "pole pairs "/1
  omega_m/1 -> pole pairs/1
  iabc_m/1 -> iabc/1
  "pole pairs "/1 -> Math Function/1
  Constant/1 -> Math Function/2
  Math Function/1 -> theta/1
  Relay/1 -> PwmON/1
  Vdc filter/1 -> Relay/1, Vdc/1
  Ifd/1 -> if/1

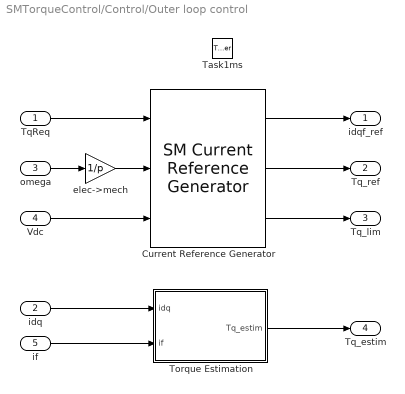
== system SMTorqueControl/Control/Outer loop control ==
  TqReq : Inport
  idq : Inport  Port=2
  omega : Inport  Port=3
  Vdc : Inport  Port=4
  if : Inport  Port=5
  Task1ms : TriggerPort  TriggerType=function-call  VariantControl=Variant  PortDimensions=1
  Current Reference Generator : eeSmCurrentReferenceGen/SM Current Reference Generator  Vnom=Vnom  Pmax=Pmax  Tmax=Tbase  ifmax=Ifbase  Ts=-1  RefType=Lookup-table based  rpmVec=RPM_VECT  TqVec=TQ_VECT  VdcVec=VDC_VECT  idMatrix=ID_MAP  iqMatrix=IQ_MAP  ifMatrix=IF_MAP  Kt=0.0375
  Torque Estimation : Subsystem
  elec->mech : Gain  Gain=1/p
  idqf_ref : Outport  VectorParamsAs1DForOutWhenUnconnected=off
  Tq_ref : Outport  Port=2  VectorParamsAs1DForOutWhenUnconnected=off
  Tq_lim : Outport  Port=3  VectorParamsAs1DForOutWhenUnconnected=off
  Tq_estim : Outport  Port=4  VectorParamsAs1DForOutWhenUnconnected=off
  wires:
  Torque Estimation/1(Tq_estim) -> Tq_estim/1
  idq/1 -> Torque Estimation/1(idq)
  if/1 -> Torque Estimation/2(if)
  Current Reference Generator/1 -> idqf_ref/1
  elec->mech/1 -> Current Reference Generator/2
  Current Reference Generator/3 -> Tq_lim/1
  Vdc/1 -> Current Reference Generator/3
  TqReq/1 -> Current Reference Generator/1
  omega/1 -> elec->mech/1
  Current Reference Generator/2 -> Tq_ref/1

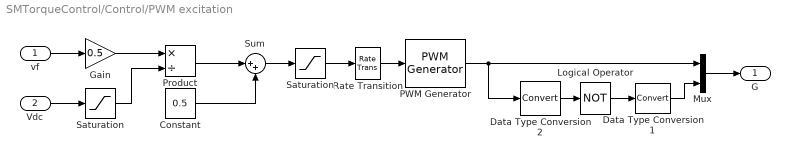
== system SMTorqueControl/Control/PWM excitation ==
  vf : Inport
  Vdc : Inport  Port=2
  Constant : Constant  Value=0.5  SampleTime=-1
  Data Type Conversion1 : DataTypeConversion  SaturateOnIntegerOverflow=off  RndMeth=Floor
  Data Type Conversion2 : DataTypeConversion  SaturateOnIntegerOverflow=off  RndMeth=Floor
  Gain : Gain  Gain=0.5
  Logical Operator : Logic  Operator=NOT  AllPortsSameDT=off  OutDataTypeStr=boolean
  Mux : Mux  Inputs=2
  PWM Generator : eePwmGenerator/PWM Generator  CarrCount=Up  Tper=1/fsw  Tdelay=0  Ts=Ts
  Product : Product  Inputs=*/
  Rate Transition : RateTransition
  Saturation : Saturate  UpperLimit=inf  LowerLimit=1
  "Saturation " : Saturate  UpperLimit=1  LowerLimit=0
  Sum : Sum  Inputs=|++
  G : Outport  VectorParamsAs1DForOutWhenUnconnected=off
  wires:
  vf/1 -> Gain/1
  Vdc/1 -> Saturation/1
  Saturation/1 -> Product/2
  Constant/1 -> Sum/2
  Sum/1 -> "Saturation "/1
  "Saturation "/1 -> Rate Transition/1
  Gain/1 -> Product/1
  Product/1 -> Sum/1
  Rate Transition/1 -> PWM Generator/1
  Data Type Conversion1/1 -> Mux/2
  PWM Generator/1 -> Data Type Conversion2/1, Mux/1
  Mux/1 -> G/1
  Data Type Conversion2/1 -> Logical Operator/1
  Logical Operator/1 -> Data Type Conversion1/1

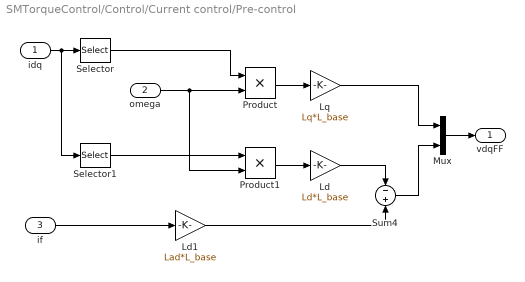
== system SMTorqueControl/Control/Current control/Pre-control ==
  idq : Inport
  omega : Inport  Port=2
  if : Inport  Port=3
  Ld : Gain  Gain=Ld*L_base
  Ld1 : Gain  Gain=Lad*L_base
  Lq : Gain  Gain=Lq*L_base
  Mux : Mux  Inputs=2
  Product : Product
  Product1 : Product
  Selector : Selector  InputPortWidth=2  IndexOptions=Index vector (dialog)  Indices=2  OutputSizes=1
  Selector1 : Selector  InputPortWidth=2  IndexOptions=Index vector (dialog)  Indices=1  OutputSizes=1
  Sum4 : Sum  Inputs=-+
  vdqFF : Outport  VectorParamsAs1DForOutWhenUnconnected=off
  wires:
  idq/1 -> Selector1/1, Selector/1
  Mux/1 -> vdqFF/1
  Selector1/1 -> Product1/1
  omega/1 -> Product1/2, Product/2
  Ld/1 -> Sum4/1
  if/1 -> Ld1/1
  Sum4/1 -> Mux/2
  Lq/1 -> Mux/1
  Ld1/1 -> Sum4/2
  Selector/1 -> Product/1
  Product1/1 -> Ld/1
  Product/1 -> Lq/1

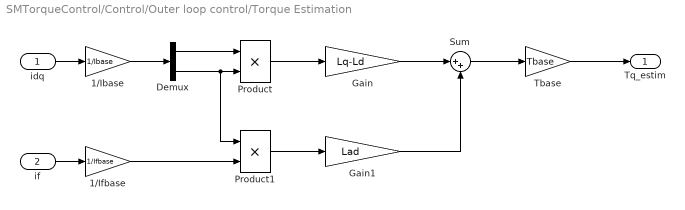
== system SMTorqueControl/Control/Outer loop control/Torque Estimation ==
  idq : Inport
  if : Inport  Port=2
  1/Ibase : Gain  Gain=1/Ibase
  1/Ifbase : Gain  Gain=1/Ifbase
  Demux : Demux  Outputs=2
  Gain : Gain  Gain=Lq-Ld
  Gain1 : Gain  Gain=Lad
  Product : Product
  Product1 : Product
  Sum : Sum  Inputs=|++
  Tbase : Gain  Gain=Tbase
  Tq_estim : Outport  VectorParamsAs1DForOutWhenUnconnected=off
  wires:
  idq/1 -> 1/Ibase/1
  Demux/1 -> Product/1
  Product/1 -> Gain/1
  Gain/1 -> Sum/1
  Demux/2 -> Product1/1, Product/2
  Product1/1 -> Gain1/1
  Sum/1 -> Tbase/1
  if/1 -> 1/Ifbase/1
  1/Ifbase/1 -> Product1/2
  1/Ibase/1 -> Demux/1
  Tbase/1 -> Tq_estim/1
  Gain1/1 -> Sum/2

== stateflow chart SMTorqueControl/Control/Task scheduler ==
  (default) -> (junction 23) : CLK_50us
  (junction 23) -> (junction 17)
  (junction 17) -> (junction 22) [order 2]
  (junction 17) -> (junction 22) [order 1] : [cnt%%2==0]{Task_100us_1;}
  (junction 22) -> (junction 18) [order 2]
  (junction 22) -> (junction 18) [order 1] : [cnt%%2==0]{Task_100us_2;}
  (junction 18) -> (junction 21) [order 1] : [cnt%%20==0]{Task_1ms_1;}
  (junction 18) -> (junction 21) [order 2]
  (junction 21) -> (junction 34) [order 2]
  (junction 21) -> (junction 16) [order 1] : [1]{cnt++;}
  data: cnt local int32
  events: Task_100us_1 output FUNCTION_CALL_EVENT; Task_100us_2 output FUNCTION_CALL_EVENT; Task_1ms_1 output FUNCTION_CALL_EVENT; CLK_50us input FUNCTION_CALL_EVENT
